simulink model "observador_continuo"  (R2023b)
settings: Solver=ode1be  StartTime=0.0  StopTime=6  FixedStep=Ts  RelTol=1e-3
values from neighbouring files (symbols this model uses):
  Ac = (T * Aa) / T    [control_moderno.m]
  Bc = T * Ba    [control_moderno.m]
  Cc = Ca / T    [control_moderno.m]
  Dc = Da    [control_moderno.m]
  Kc = place(Ac,Bc,polyc)    [control_moderno.m]
  Lc = acker(Ac.',Cc.',polyec).'    [control_moderno.m]
libraries: cstblocks x1
settings Model: Creator=aghersin  LastModifiedBy=agust
settings SolverCC: AlgebraicLoopSolver=TrustRegion
settings DataIOCC: ReturnWorkspaceOutputs=off
settings DebuggingCC: UnconnectedInputMsg=warning  UnconnectedOutputMsg=warning  UnconnectedLineMsg=warning  ArithmeticOperatorsInVariantConditions=warning
settings ModelReferenceCC: EnableRefExpFcnMdlSchedulingChecks=on
settings SFSimCC: SimUseLocalCustomCode=off  CustomCodeUndefinedFunction=UseInterfaceOnly
settings RTWCC: RTWUseLocalCustomCode=off

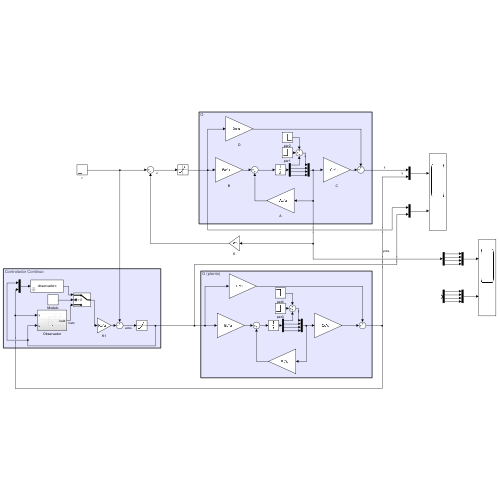
[thumbnail: Simulink's stored preview of the top-level diagram]
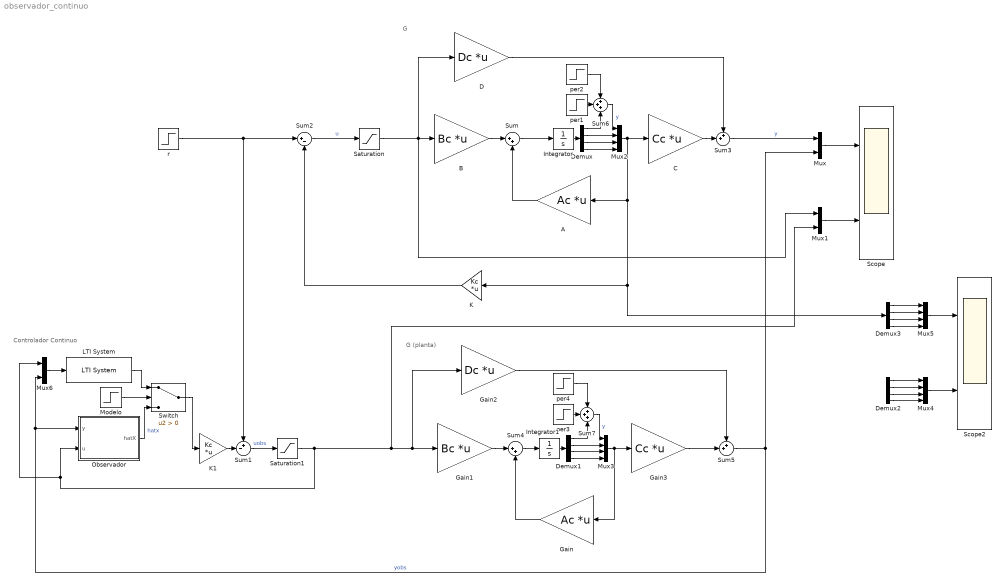
== system observador_continuo ==
  note: Controlador Continuo
  note: G (planta)
  note: G
  A : Gain  Gain=Ac  Multiplication=Matrix(K*u)
  B : Gain  Gain=Bc  Multiplication=Matrix(K*u)
  C : Gain  Gain=Cc  Multiplication=Matrix(K*u)
  D : Gain  Gain=Dc  Multiplication=Matrix(K*u)
  Demux{,1..3} (4 alike) : Demux
  Gain : Gain  Gain=Ac  Multiplication=Matrix(K*u)
  Gain1 : Gain  Gain=Bc  Multiplication=Matrix(K*u)
  Gain2 : Gain  Gain=Dc  Multiplication=Matrix(K*u)
  Gain3 : Gain  Gain=Cc  Multiplication=Matrix(K*u)
  Integrator : Integrator  InitialCondition=[0, 0, 0, 0]
  Integrator1 : Integrator  InitialCondition=[0, 0, 0, 0]
  K : Gain  Gain=Kc  Multiplication=Matrix(K*u)
  K1 : Gain  Gain=Kc  Multiplication=Matrix(K*u)
  LTI System : cstblocks/LTI System  sys=observadorc  IC=[]  PadeOrder=0
  Modelo : Step  Time=0.5  After=-1  SampleTime=0
  Mux : Mux  Inputs=2
  Mux1 : Mux  Inputs=2
  Mux{2..5} (4 alike) : Mux
  Mux6 : Mux  Inputs=2
  Observador : Subsystem
  Saturation : Saturate  UpperLimit=30  LowerLimit=-30
  Saturation1 : Saturate  UpperLimit=30  LowerLimit=-30
  Scope : Scope  NumInputPorts=2
  Scope2 : Scope  NumInputPorts=2
  Sum : Sum  Inputs=|++
  Sum1 : Sum  Inputs=+-|
  Sum2 : Sum  Inputs=|+-
  Sum3 : Sum  Inputs=++|
  Sum4 : Sum  Inputs=|++
  Sum5 : Sum  Inputs=++|
  Sum6 : Sum  Inputs=+++
  Sum7 : Sum  Inputs=+++
  Switch : Switch  Criteria=u2 > Threshold  SaturateOnIntegerOverflow=off  InputSameDT=off
  per1 : Step  After=30  SampleTime=0
  per2 : Step  Time=1.1  After=-30  SampleTime=0
  per3 : Step  After=30  SampleTime=0
  per4 : Step  Time=1.1  After=-30  SampleTime=0
  r : Step  After=0  SampleTime=0
  wires:
  K/1 -> Sum2/2
  Sum2/1 -> Saturation/1  "u"
  Sum3/1 -> Mux/1  "y"
  Sum5/1 -> Mux/2, Mux6/2, Observador/1(y)  "yobs"
  Mux/1 -> Scope/1
  Mux1/1 -> Scope/2
  B/1 -> Sum/1
  A/1 -> Sum/2
  D/1 -> Sum3/1
  Sum/1 -> Integrator/1
  C/1 -> Sum3/2
  Gain3/1 -> Sum5/2
  Gain2/1 -> Sum5/1
  Gain/1 -> Sum4/2
  Gain1/1 -> Sum4/1
  Sum1/1 -> Saturation1/1  "uobs"
  r/1 -> Sum1/1, Sum2/1
  K1/1 -> Sum1/2
  Integrator/1 -> Demux/1
  Mux2/1 -> A/1, Demux3/1, K/1, C/1
  per1/1 -> Sum6/2
  per2/1 -> Sum6/1
  Demux/2 -> Mux2/2
  Demux/3 -> Mux2/3
  Demux/4 -> Mux2/4
  Sum6/1 -> Mux2/1  "y"
  Demux/1 -> Sum6/3
  per4/1 -> Sum7/1
  Integrator1/1 -> Demux1/1
  per3/1 -> Sum7/2
  Demux1/1 -> Sum7/3
  Sum4/1 -> Integrator1/1
  Mux3/1 -> Gain3/1, Gain/1
  Sum7/1 -> Mux3/1  "y"
  Demux1/2 -> Mux3/2
  Demux1/3 -> Mux3/3
  Demux1/4 -> Mux3/4
  Saturation/1 -> D/1, Mux1/1, B/1
  Saturation1/1 -> Observador/2(u), Mux6/1, Mux1/2, Gain1/1, Gain2/1
  Demux2/4 -> Mux4/4
  Demux2/1 -> Mux4/1
  Demux2/2 -> Mux4/2
  Demux2/3 -> Mux4/3
  Mux4/1 -> Scope2/2
  Mux5/1 -> Scope2/1
  Demux3/3 -> Mux5/3
  Demux3/4 -> Mux5/4
  Demux3/2 -> Mux5/2
  Demux3/1 -> Mux5/1
  Mux6/1 -> LTI System/1
  Switch/1 -> K1/1
  LTI System/1 -> Switch/1
  Observador/1(hatX) -> Switch/3  "hatx"
  Modelo/1 -> Switch/2

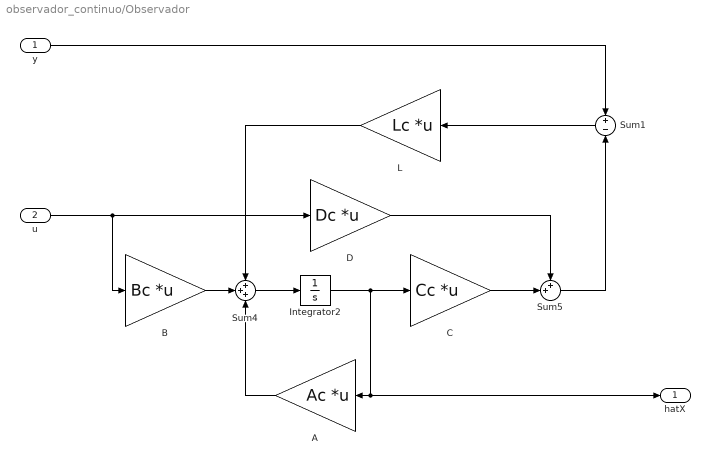
== system observador_continuo/Observador ==
  y : Inport
  u : Inport  Port=2
  A : Gain  Gain=Ac  Multiplication=Matrix(K*u)
  B : Gain  Gain=Bc  Multiplication=Matrix(K*u)
  C : Gain  Gain=Cc  Multiplication=Matrix(K*u)
  D : Gain  Gain=Dc  Multiplication=Matrix(K*u)
  Integrator2 : Integrator
  L : Gain  Gain=Lc  Multiplication=Matrix(K*u)
  Sum1 : Sum  Inputs=+|-
  Sum4 : Sum  Inputs=+++
  Sum5 : Sum  Inputs=++|
  hatX : Outport  VectorParamsAs1DForOutWhenUnconnected=off
  wires:
  L/1 -> Sum4/1
  A/1 -> Sum4/3
  B/1 -> Sum4/2
  u/1 -> D/1, B/1
  Sum4/1 -> Integrator2/1
  C/1 -> Sum5/2
  D/1 -> Sum5/1
  Sum1/1 -> L/1
  Integrator2/1 -> C/1, hatX/1, A/1
  Sum5/1 -> Sum1/2
  y/1 -> Sum1/1
